simulink model "CruiseFuzzy"  (R2024a)
settings: Solver=ode4  StartTime=0.0  StopTime=30  FixedStep=1e-3  RelTol=1e-3
PreLoadFcn:
  | cc_init;
values from neighbouring files (symbols this model uses):
  p = cc_params()    [cc_init.m]    (also in cc_run.m; cc_sim.m)
libraries: fuzblock x1
settings Model: Creator=27812  LastModifiedBy=27812

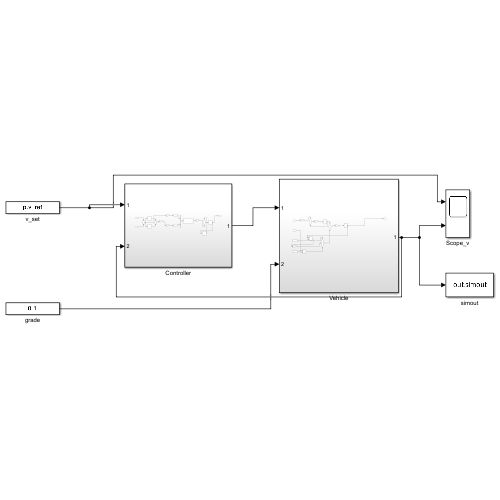
[thumbnail: Simulink's stored preview of the top-level diagram]
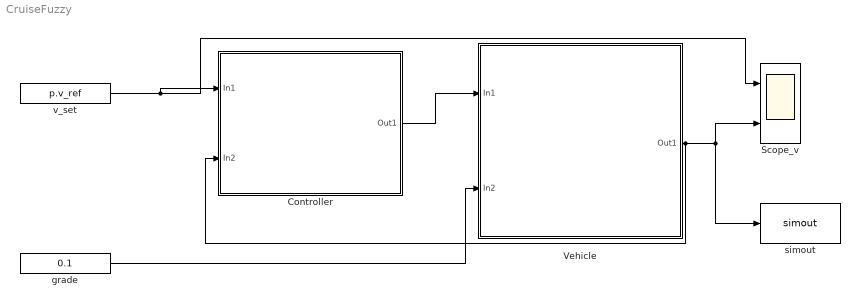
== system CruiseFuzzy ==
  Controller : Subsystem
  Scope_v : Scope  NumInputPorts=2
  Vehicle : Subsystem
  grade : Constant  Value=0.1
  simout : ToWorkspace  VariableName=simout  SaveFormat=Structure With Time  SampleTime=-1
  v_set : Constant  Value=p.v_ref
  wires:
  v_set/1 -> Controller/1(In1), Scope_v/1
  grade/1 -> Vehicle/2(In2)
  Controller/1(Out1) -> Vehicle/1(In1)
  Vehicle/1(Out1) -> Scope_v/2, simout/1, Controller/2(In2)

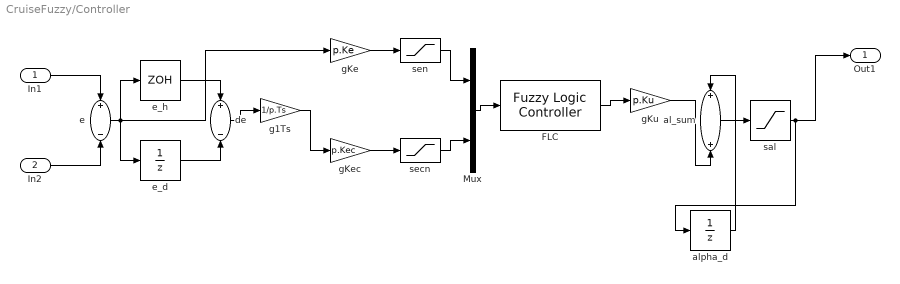
== system CruiseFuzzy/Controller ==
  In1 : Inport
  In2 : Inport  Port=2
  FLC : fuzblock/Fuzzy Logic  Controller  FIS=cruise_fuzzy  OutputSampleNumber=101  DataType=double  FuzzifiedInputs=off  RuleFiringStrengths=off  RuleOutputs=off  AggregatedOutputs=off  SimulateUsing=Interpreted execution  OutOfRangeInputValueMessage=warning  NoRuleFiredMessage=warning  EmptyOutputFuzzySetMessage=warning
  Mux : Mux  Inputs=2
  al_sum : Sum
  alpha_d : UnitDelay  InitialCondition=p.alpha0  SampleTime=p.Ts  HasFrameUpgradeWarning=on
  de : Sum  Inputs=+-
  e : Sum  Inputs=+-
  e_d : UnitDelay  SampleTime=p.Ts  HasFrameUpgradeWarning=on
  e_h : ZeroOrderHold  SampleTime=p.Ts
  g1Ts : Gain  Gain=1/p.Ts
  gKe : Gain  Gain=p.Ke
  gKec : Gain  Gain=p.Kec
  gKu : Gain  Gain=p.Ku
  sal : Saturate  UpperLimit=1  LowerLimit=0
  secn : Saturate  UpperLimit=1  LowerLimit=-1
  sen : Saturate  UpperLimit=1  LowerLimit=-1
  Out1 : Outport
  wires:
  In1/1 -> e/1
  In2/1 -> e/2
  e/1 -> e_h/1, e_d/1, gKe/1
  e_h/1 -> de/1
  e_d/1 -> de/2
  de/1 -> g1Ts/1
  g1Ts/1 -> gKec/1
  gKec/1 -> secn/1
  secn/1 -> Mux/2
  gKe/1 -> sen/1
  sen/1 -> Mux/1
  Mux/1 -> FLC/1
  FLC/1 -> gKu/1
  gKu/1 -> al_sum/2
  alpha_d/1 -> al_sum/1
  al_sum/1 -> sal/1
  sal/1 -> Out1/1, alpha_d/1

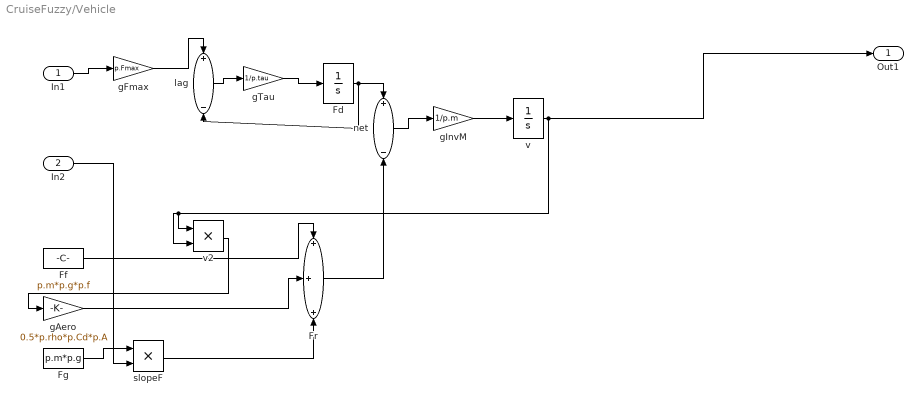
== system CruiseFuzzy/Vehicle ==
  In1 : Inport
  In2 : Inport  Port=2
  Fd : Integrator  InitialCondition=p.Fd0
  Ff : Constant  Value=p.m*p.g*p.f
  Fg : Constant  Value=p.m*p.g
  Fr : Sum  Inputs=+++
  gAero : Gain  Gain=0.5*p.rho*p.Cd*p.A
  gFmax : Gain  Gain=p.Fmax
  gInvM : Gain  Gain=1/p.m
  gTau : Gain  Gain=1/p.tau
  lag : Sum  Inputs=+-
  net : Sum  Inputs=+-
  slopeF : Product  Inputs=**
  v : Integrator  InitialCondition=p.v_ref
  v2 : Product  Inputs=**
  Out1 : Outport
  wires:
  In1/1 -> gFmax/1
  gFmax/1 -> lag/1
  Fd/1 -> lag/2, net/1
  lag/1 -> gTau/1
  gTau/1 -> Fd/1
  v/1 -> v2/1, v2/2, Out1/1
  v2/1 -> gAero/1
  gAero/1 -> Fr/2
  Ff/1 -> Fr/1
  Fg/1 -> slopeF/1
  In2/1 -> slopeF/2
  slopeF/1 -> Fr/3
  Fr/1 -> net/2
  net/1 -> gInvM/1
  gInvM/1 -> v/1
